simulink model "bev_motor_cooling"  (R2025a)
settings: Solver=VariableStepAuto  StartTime=0.0  StopTime=720  RelTol=1e-3  AbsTol=1e-3
PreLoadFcn:
  | bev_motor_cooling_param;
undefined symbols (not defined in the file): bev
libraries: fl_lib x24, SimscapeFluids_lib x4, nesl_utility x4, driver_maneuver_library x1, ee_lib x1, sdl_lib x1
CloseFcn:
  | try,close(h1_bev_motor_cooling),end
  | clear h1_bev_motor_cooling
  | try,close(h2_bev_motor_cooling),end
  | clear h2_bev_motor_cooling
  | try,close(h3_bev_motor_cooling),end
  | clear h3_bev_motor_cooling
  | try,close(h4_bev_motor_cooling),end
  | clear h4_bev_motor_cooling
  | 
  | 
  | clear simlog_bev_motor_cooling
  | clear logsout_bev_motor_cooling
Description:
  | Battery Electric Vehicle With Motor Cooling
  | 
  | 
  | Copyright 2021-2025 The MathWorks, Inc.
settings Model: Creator=kheintz  LastModifiedBy=smiller
settings SolverCC: AutoScaleAbsTol=off  AlgebraicLoopSolver=TrustRegion
settings DataIOCC: MaxDataPoints=10000  SignalLoggingName=logsout_bev_motor_cooling
settings OptimizationCC: ReuseModelBlockBuffer=off
settings DebuggingCC: UnconnectedInputMsg=warning  UnconnectedOutputMsg=warning  UnconnectedLineMsg=warning  SymbolicDimsDataTypeCodeGenerationDiagnostic=none
settings ModelReferenceCC: EnableRefExpFcnMdlSchedulingChecks=on
settings SFSimCC: CustomCodeUndefinedFunction=UseInterfaceOnly
settings RTWCC: GPUComputeCapability=3.5  DLArmComputeVersion=19.05
settings SimscapeCC: SimscapeLogType=all  SimscapeLogSimulationStatistics=on  SimscapeLogName=simlog_bev_motor_cooling  SimscapeLogDataHistory=10000.0

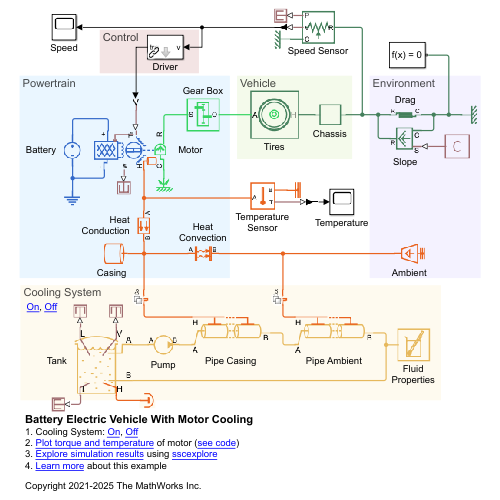
[thumbnail: Simulink's stored preview of the top-level diagram]
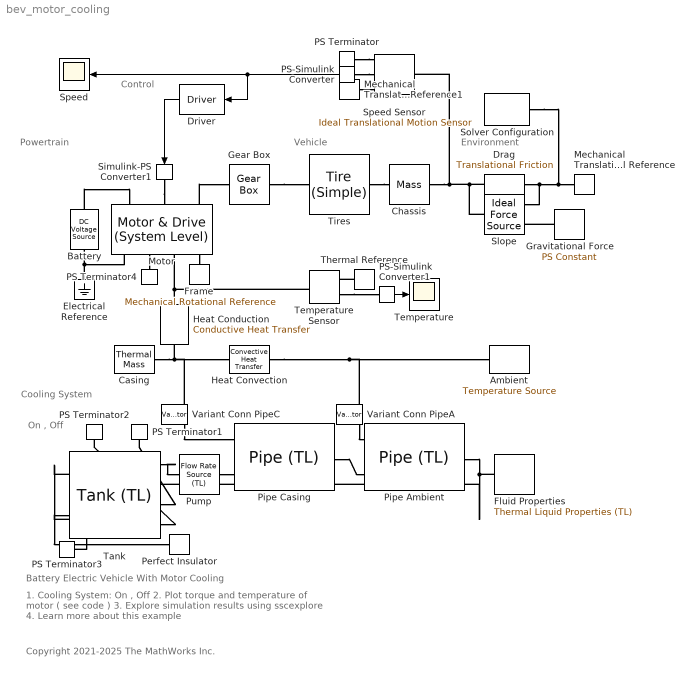
== system bev_motor_cooling ==
  note: Copyright 2021-2025 The MathWorks Inc.
  note: Control
  note: Environment
  note: Powertrain
  note: Vehicle
  note: Cooling System
  note: Battery Electric Vehicle With Motor Cooling
  note: 1. Cooling System: On , Off
      | 2. Plot torque and temperature of motor ( see code )
      | 3. Explore simulation results using sscexplore
      | 4. Learn more about this example
  note: On , Off
  Ambient : fl_lib/Thermal/Thermal Sources/Temperature Source  temperature=bev.Tambient degC
  Battery : fl_lib/Electrical/Electrical Sources/DC Voltage Source  v0=bev.battery.volt V
  Casing : fl_lib/Thermal/Thermal Elements/Thermal Mass  mass_type=foundation.enum.constant_variable.constant  mass=bev.casing.mass kg  sp_heat=bev.casing.sp_heat J/kg/K  mass_min=1e-6 kg  num_ports=foundation.enum.numPorts2.one  m_specify=off  m_priority=High  m=1 kg  m_nominal_specify=off  m_nominal_value=1  m_nominal_unit=kg  T_specify=on  T_priority=High  T=bev.casing.initT degC  T_nominal_specify=off  T_nominal_value=1  T_nominal_unit=K  Q_specify=off  Q_priority=None  Q=0 W  Q_nominal_specify=off  Q_nominal_value=1  Q_nominal_unit=W
  Chassis : fl_lib/Mechanical/Translational Elements/Mass  mass=bev.car.mass kg  num_ports=foundation.enum.numPorts2.two  v_specify=off  v_priority=Low  v=100 km/hr  v_nominal_specify=off  v_nominal_value=10  v_nominal_unit=m/s  f_specify=off  f_priority=None  f=0 N  f_nominal_specify=off  f_nominal_value=1  f_nominal_unit=N
      settings: InternalSimscapePortConfiguration="{\"Bottom\":[],\"Left\":[{\"id\":\"M\",\"label\":\"\",\"type\":\"foundation.mechanical.translational.translational\"}],\"Right\":[{\"id\":\"N\",\"label\":\"\",\"type\":\"foundation.mechanical.translational.translational\"}],\"Top\":[]}"
  Drag : fl_lib/Mechanical/Translational Elements/Translational Friction  brkwy_frc=bev.car.drag.brk N  brkwy_vel=bev.car.drag.vth m/s  Col_frc=bev.car.drag.fcl N  visc_coef=bev.car.drag.cvs N/(m/s)  v_specify=off  v_priority=None  v=0 m/s  v_nominal_specify=off  v_nominal_value=1  v_nominal_unit=m/s  f_specify=off  f_priority=None  f=0 N  f_nominal_specify=off  f_nominal_value=1  f_nominal_unit=N
      settings: InternalSimscapePortConfiguration="{\"Bottom\":[],\"Left\":[{\"id\":\"R\",\"label\":\"R\",\"type\":\"foundation.mechanical.translational.translational\"}],\"Right\":[{\"id\":\"C\",\"label\":\"C\",\"type\":\"foundation.mechanical.translational.translational\"}],\"Top\":[]}"
  Driver : driver_maneuver_library/Driver  max_torque=800  spd_cruise_1=100  spd_other_car=80  initial_lead_dist=100  follow_dist=40  pass_start_time=180  spd_passing=160  lead_dist=20  spd_cruise_2=100
  Electrical Reference : fl_lib/Electrical/Electrical Elements/Electrical Reference
  Fluid Properties : SimscapeFluids_lib/Thermal Liquid/Utilities/Thermal Liquid Properties (TL)  fluid_list=fluids.thermal_liquid.utilities.enum.thermal_liquid_fluid_list.ethylene_glycol  concentration_param_EG=fluids.thermal_liquid.utilities.enum.thermal_liquid_concentration.volume_fraction  concentration_param_PG=fluids.thermal_liquid.utilities.enum.thermal_liquid_concentration.volume_fraction  c_mass_SW=3.5e-3  c_mass_EG=0.1  c_mass_PG=0.1  c_mass_GL=0.1  c_vol_EG=0.5  c_vol_PG=0.1  beta_const_EG=2.1791 GPa  beta_const_PG=2.1791 GPa  beta_const_GL=2.1791 GPa  p_min_EG=0.01 MPa  p_min_PG=0.01 MPa  p_min_GL=0.01 MPa  p_max_EG=50 MPa  p_max_PG=50 MPa  p_max_GL=50 MPa  p_atm=0.101325 MPa  properties_range_check=simscape.enum.assert.action.error
  Frame : fl_lib/Mechanical/Rotational Elements/Mechanical Rotational Reference
  Gear Box : fl_lib/Mechanical/Mechanisms/Gear Box  Tag=varswap  ratio=bev.car.gear.rat  t_in_specify=off  t_in_priority=None  t_in=0 N*m  t_in_nominal_specify=off  t_in_nominal_value=1  t_in_nominal_unit=N*m  t_out_specify=off  t_out_priority=None  t_out=0 N*m  t_out_nominal_specify=off  t_out_nominal_value=1  t_out_nominal_unit=N*m
  Gravitational Force : fl_lib/Physical Signals/Sources/PS Constant  constant=bev.road.gforce N
  Heat Conduction : fl_lib/Thermal/Thermal Elements/Conductive Heat Transfer  thermal_type=foundation.enum.ConstantVariableTabulated.Constant  wall_geometry=foundation.enum.ConductionWallGeometry.Planar  area=bev.motor.qcond.area m^2  thickness=bev.motor.qcond.thick m  d_in=0.05 m  d_out=0.1 m  L=1 m  th_cond_min=10 W/(K*m)  th_cond=bev.motor.qcond.th_cond W/(m*K)  th_cond_TLU=[413, 401, 392, 383, 371, 357, 342] W/(K*m)  temp_TLU=[200, 273, 400, 600, 800, 1000, 1200] K  T_specify=off  T_priority=None  T=0 K  T_nominal_specify=off  T_nominal_value=1  T_nominal_unit=K  Q_specify=off  Q_priority=None  Q=1 W  Q_nominal_specify=off  Q_nominal_value=1  Q_nominal_unit=W
  Heat Convection : fl_lib/Thermal/Thermal Elements/Convective Heat Transfer  thermal_type=foundation.enum.constant_variable.constant  area=bev.casing.qconv.area m^2  heat_tr_coeff=bev.casing.qconv.th_conv W/(m^2 * K)  min_heat_tr_coeff=1e-3 W/(K*m^2)  T_specify=off  T_priority=None  T=0 K  T_nominal_specify=off  T_nominal_value=1  T_nominal_unit=K  Q_specify=off  Q_priority=None  Q=0 W  Q_nominal_specify=off  Q_nominal_value=1  Q_nominal_unit=W
  Mechanical Translational Reference : fl_lib/Mechanical/Translational Elements/Mechanical Translational Reference
  Mechanical Translational Reference1 : fl_lib/Mechanical/Translational Elements/Mechanical Translational Reference
  Motor : ee_lib/Electromechanical/Motor & Drive (System Level)  torque_speed_param=ee.enum.electromech.envelope.torque_power  overtorque_param=ee.enum.electromech.overtorque.no  T_t=[.09, .08, .07, 0] N*m  T_t_intermittent=[.36, .32, .28, 0] N*m  T_t_2D=[.09, .09, .09; .08, .08, .08; .07, .07, .07; 0, 0, 0] N*m  T_t_intermittent_2D=[.36, .36, .36; .32, .32, .32; .28, .28, .28; 0, 0, 0] N*m  w_t=[0, 3750, 7500, 8000] rpm  vdc_t=[6, 12, 24] V  torque_max=bev.motor.maxtrq N*m  power_max=bev.motor.maxpwr W  torque_max_intermittent=0.4 N*m  power_max_intermittent=120 W  time_overtorque=30 s  time_recover=60 s  Tc=bev.motor.tc s  EnableSwitch=simscape.enum.onoff.off  losses_param=1  eff=bev.motor.eff  w_eff=bev.motor.w_eff rpm  T_eff=bev.motor.T_eff N*m  Piron=bev.motor.Piron W  Pbase=bev.motor.Pbase W  w_eff_vec=[-8000, -4000, 0, 4000, 8000] rpm  T_eff_vec=[0, .03, .06, .09] N*m  v_eff_vec=[100, 250, 400] V  losses_mat=[1.49, 1.67, 2.21, 3.1; .42, .69, 1.14, 2.03; .06, .24, .78, 1.68; .42, .69, 1.14, 2.03; 1.49, 1.67, 2.21, 3.1] W  efficiency_mat=[95, 95, 95, 95; 95, 95, 95, 95; 95, 95, 95, 95; 95, 95, 95, 95; 95, 95, 95, 95]  losses_mat_3D=ones(5, 4, 3) W  efficiency_mat_3D=95 * ones(5, 4, 3)  Res=bev.motor.Res Ohm  J=bev.motor.J kg*m^2  lam=bev.motor.lam N*m/(rad/s)  speed0=bev.motor.speed0 rpm  faulted_specify=off  faulted_priority=None  faulted=0  faulted_nominal_specify=off  faulted_nominal_value=1  faulted_nominal_unit=1  isSwitchedOff_specify=off  isSwitchedOff_priority=None  isSwitchedOff=0  isSwitchedOff_nominal_specify=off  isSwitchedOff_nominal_value=1  isSwitchedOff_nominal_unit=1  torqueLimitContinuous_specify=off  torqueLimitContinuous_priority=None  torqueLimitContinuous=0 N*m  torqueLimitContinuous_nominal_specify=off  torqueLimitContinuous_nominal_value=1  torqueLimitContinuous_nominal_unit=N*m  alpha=bev.motor.alpha 1/K  Tmeas=bev.motor.Tmeas degC  Tmeas2=125 degC  losses_mat_T2=[1.49, 1.74, 2.49, 3.74; .42, .67, 1.42, 2.67; .06, .31, 1.06, 2.31; .42, .67, 1.42, 2.67; 1.49, 1.74, 2.49, 3.74] W  efficiency_mat_T2=[95, 95, 95, 95; 95, 95, 95, 95; 95, 95, 95, 95; 95, 95, 95, 95; 95, 95, 95, 95]  losses_mat_3D_T2=ones(5, 4, 3) W  efficiency_mat_3D_T2=95 * ones(5, 4, 3)  thermal_mass=bev.motor.thermal_mass J/K  initial_temperature=bev.motor.initT degC
      settings: InternalSimscapePortConfiguration="{\"Bottom\":[],\"Left\":[{\"id\":\"Vp\",\"label\":\"+\",\"type\":\"foundation.electrical.electrical\"},{\"id\":\"Tr\",\"label\":\"Tr\",\"type\":\"input\"},{\"id\":\"R\",\"label\":\"R\",\"type\":\"foundation.mechanical.rotational.rotational\"}],\"Right\":[{\"id\":\"Vm\",\"label\":\"-\",\"type\":\"foundation.electrical.electrical\"},{\"id\":\"Omega\",\"label\":\"w\",\"type\":\"output\"},{\"id\":\"H\",\"label\":\"H\",\"type\":\"foundation.thermal.thermal\"},{\"id\":\"C\",\"label\":\"C\",\"type\":\"foundation.mechanical.rotational.rotational\"}],\"Top\":[]}"
  PS Terminator{,1..4} (5 alike) : fl_lib/Physical Signals/Sinks/PS Terminator
  PS-Simulink Converter : nesl_utility/PS-Simulink Converter  PhysicalDomain=network_engine_domain  SubClassName=ps_output  LeftPortType=input  RightPortType=output  PseudoPeriodic=off  Frequencies=[]  VectorFormat=1-D array  Unit=km/hr  AffineConversion=off
  PS-Simulink Converter1 : nesl_utility/PS-Simulink Converter  PhysicalDomain=network_engine_domain  SubClassName=ps_output  LeftPortType=input  RightPortType=output  PseudoPeriodic=off  Frequencies=[]  VectorFormat=1-D array  Unit=degC  AffineConversion=on
  Perfect Insulator : fl_lib/Thermal/Thermal Elements/Perfect Insulator  T_specify=off  T_priority=None  T=0 K  T_nominal_specify=off  T_nominal_value=1  T_nominal_unit=K
  Pipe Ambient : SimscapeFluids_lib/Thermal Liquid/Pipes & Fittings/Pipe (TL)  dynamic_compressibility=1  inertia=0  num_segments=10  pipe_length=5 m  cross_section_geometry=fluids.thermal_liquid.pipes_fittings.enum.CrossSectionGeometry.Custom  pipe_diameter=0.1 m  pipe_inner_diameter=0.05 m  pipe_outer_diameter=0.1 m  pipe_width=0.1 m  pipe_height=0.1 m  pipe_major_axis=0.1 m  pipe_minor_axis=0.05 m  pipe_side=0.1 m  pipe_angle=30 deg  area=bev.cooling.area m^2  Dh=bev.cooling.hd m  elevation_spec=foundation.enum.constant_variable.constant  elevation_gain=0 m  gravity_spec=foundation.enum.constant_variable.constant  g=9.81 m/s^2  pressure_loss_spec=1  local_pressure_loss_spec=fluids.thermal_liquid.pipes_fittings.enum.LocalLossSpec.AggregateLength  length_add=1 m  loss_coefficient=0.1  roughness_spec=fluids.thermal_liquid.pipes_fittings.enum.RoughnessSpec.Custom  roughness=1.5e-5 m  Re_friction_TLU=[ 400 1000 1.5e+3 3e+3 4e+3 6e+3 1e+4 2e+4 4e+4 6e+4 1e+5 1e+8 ]  friction_factor_TLU=[ 0.264 0.112 0.07099999999999999 0.0417 0.0387 0.0268 0.025 0.0232 0.0226 0.022 0.0214 0.0214 ]  Re_lam=2e+3  Re_tur=4e+3  shape_factor=64  mdot_nominal=[ 0.1 1 ] kg/s  p_diff_nominal=[ 0.001 0.01 ] MPa  mdot_threshold=1e-6 kg/s  wall_spec=1  vol_expansion_spec=fluids.thermal_liquid.pipes_fittings.enum.VolumeExpansionSpec.Diameter  area_pressure_gain=1e-6 m^2/MPa  static_pressure_TLU=[.1, 1] MPa  area_pressure_gain_TLU=[1e-05, 1.1e-05] m^2  material_behavior_spec=fluids.thermal_liquid.pipes_fittings.enum.PipeMaterialBehavior.Linear  diameter_pressure_gain=1.2e-6 m/MPa  wall_thickness=0.05 m  elastic_modulus=69 GPa  stress_TLU=[276, 310] MPa  strain_TLU=[.004, .02]  stress_assert_action=simscape.enum.assert.action.none  stress_max=400 MPa  poisson_ratio=0.33  wall_time_constant=0.01 s  thermal_expansion=false  alpha_L_wall=24 um/(deltaK*m)  thermal_expansion_Tref=293.15 K  heat_transfer_spec=1  mdot_nominal_heat=[ 0.1 1 ] kg/s  T_in_nominal=[ 293.15 293.15 ] K  T_out_nominal=[ 300 300 ] K  p_in_nominal_heat=[ 0.101325 0.101325 ] MPa  T_wall_nominal=[ 303.15 303.15 ] K  a_coeff=0.023  b_Re_power=0.8  c_Pr_power=0.4  Nu_lam=3.66  Re_Colburn_TLU=[ 100 150 1000 ]  Colburn_factor_TLU=[ 0.019 0.013 0.002 ]  Re_Nu_TLU=[ 100 150 1000 ]  Pr_Nu_TLU=[ 1 10 ]  Nu_TLU=[ 3.72 4.21; 3.75 4.44; 4.21 7.15 ]  p0_vec=0.101325 MPa  T0_vec=bev.Tambient degC  mdot0=0.1 kg/s  p_nominal=0.101325 MPa  T_nominal=293.15 K
  Pipe Casing : SimscapeFluids_lib/Thermal Liquid/Pipes & Fittings/Pipe (TL)  dynamic_compressibility=1  inertia=0  num_segments=10  pipe_length=5 m  cross_section_geometry=fluids.thermal_liquid.pipes_fittings.enum.CrossSectionGeometry.Custom  pipe_diameter=0.1 m  pipe_inner_diameter=0.05 m  pipe_outer_diameter=0.1 m  pipe_width=0.1 m  pipe_height=0.1 m  pipe_major_axis=0.1 m  pipe_minor_axis=0.05 m  pipe_side=0.1 m  pipe_angle=30 deg  area=bev.cooling.area m^2  Dh=bev.cooling.hd m  elevation_spec=foundation.enum.constant_variable.constant  elevation_gain=0 m  gravity_spec=foundation.enum.constant_variable.constant  g=9.81 m/s^2  pressure_loss_spec=1  local_pressure_loss_spec=fluids.thermal_liquid.pipes_fittings.enum.LocalLossSpec.AggregateLength  length_add=1 m  loss_coefficient=0.1  roughness_spec=fluids.thermal_liquid.pipes_fittings.enum.RoughnessSpec.Custom  roughness=1.5e-5 m  Re_friction_TLU=[ 400 1000 1.5e+3 3e+3 4e+3 6e+3 1e+4 2e+4 4e+4 6e+4 1e+5 1e+8 ]  friction_factor_TLU=[ 0.264 0.112 0.07099999999999999 0.0417 0.0387 0.0268 0.025 0.0232 0.0226 0.022 0.0214 0.0214 ]  Re_lam=2e+3  Re_tur=4e+3  shape_factor=64  mdot_nominal=[ 0.1 1 ] kg/s  p_diff_nominal=[ 0.001 0.01 ] MPa  mdot_threshold=1e-6 kg/s  wall_spec=1  vol_expansion_spec=fluids.thermal_liquid.pipes_fittings.enum.VolumeExpansionSpec.Diameter  area_pressure_gain=1e-6 m^2/MPa  static_pressure_TLU=[.1, 1] MPa  area_pressure_gain_TLU=[1e-05, 1.1e-05] m^2  material_behavior_spec=fluids.thermal_liquid.pipes_fittings.enum.PipeMaterialBehavior.Linear  diameter_pressure_gain=1.2e-6 m/MPa  wall_thickness=0.05 m  elastic_modulus=69 GPa  stress_TLU=[276, 310] MPa  strain_TLU=[.004, .02]  stress_assert_action=simscape.enum.assert.action.none  stress_max=400 MPa  poisson_ratio=0.33  wall_time_constant=0.01 s  thermal_expansion=false  alpha_L_wall=24 um/(deltaK*m)  thermal_expansion_Tref=293.15 K  heat_transfer_spec=1  mdot_nominal_heat=[ 0.1 1 ] kg/s  T_in_nominal=[ 293.15 293.15 ] K  T_out_nominal=[ 300 300 ] K  p_in_nominal_heat=[ 0.101325 0.101325 ] MPa  T_wall_nominal=[ 303.15 303.15 ] K  a_coeff=0.023  b_Re_power=0.8  c_Pr_power=0.4  Nu_lam=3.66  Re_Colburn_TLU=[ 100 150 1000 ]  Colburn_factor_TLU=[ 0.019 0.013 0.002 ]  Re_Nu_TLU=[ 100 150 1000 ]  Pr_Nu_TLU=[ 1 10 ]  Nu_TLU=[ 3.72 4.21; 3.75 4.44; 4.21 7.15 ]  p0_vec=0.101325 MPa  T0_vec=bev.casing.initT degC  mdot0=0.1 kg/s  p_nominal=0.101325 MPa  T_nominal=293.15 K
  Pump : fl_lib/Thermal Liquid/Sources/Flow Rate Source (TL)  source_type=foundation.enum.constant_controlled.constant  flow_type=foundation.enum.mass_volumetric_flow.mass  mass_flow=2 kg/s  volumetric_flow=0 m^3/s  power_spec=foundation.enum.power_spec.isentropic  area=0.01 m^2
      settings: InternalSimscapePortConfiguration="{\"Bottom\":[],\"Left\":[{\"id\":\"A\",\"label\":\"A\",\"type\":\"foundation.thermal_liquid.thermal_liquid\"}],\"Right\":[{\"id\":\"B\",\"label\":\"B\",\"type\":\"foundation.thermal_liquid.thermal_liquid\"}],\"Top\":[]}"
  Simulink-PS Converter1 : nesl_utility/Simulink-PS Converter  PhysicalDomain=network_engine_domain  SubClassName=ps_input  LeftPortType=input  RightPortType=output  PseudoPeriodic=off  Frequencies=[]  NoiseDistribution=none  NoiseParameters=[]  Unit=N*m  AffineConversion=off  FilteringAndDerivatives=provide  SimscapeFilterOrder=1  InputFilterTimeConstant=0.001  UdotUserProvided=0
  Slope : fl_lib/Mechanical/Mechanical Sources/Ideal Force Source
  Solver Configuration : nesl_utility/Solver Configuration  PhysicalDomain=network_engine_domain  SubClassName=solver  LeftPortType=input  RightPortType=generic  Tones=[]  Harmonics=[]  SimulateNoise=off  Profile=off  UseLocalSampling=off  EnableSwitchedLinearOptims=on  FrequencyDomain=off  UseCCode=off  RelTol=0.001  AbsTol=1e-06  MinStep=1e-09  ToWorkspace=off  RevertToSquareIcSolve=off  NumHomotopyIterations=100  PhasorMode=off  PhasorModeNumHarmonics=1  ConsistencySolver=NEWTON_FTOL  IndexReductionMethod=DerivativeReplacement  DoDC=off  ResidualTolerance=1e-09  ConsistencyTolSource=GLOBAL  ConsistencyAbsTol=0.001  ConsistencyRelTol=0.001  ConsistencyTolFactor=0.001  UseLocalSolver=off  LocalSolverChoice=NE_BACKWARD_EULER_ADVANCER  ResolveIndetEquations=on  FunctionEvalNumThread=1  LocalSolverSampleTime=0.001  DoFixedCost=off  MaxNonlinIter=3  MaxModeIter=2  ComputeImpulses=off  ImpulseIterations=2  LinearAlgebra=auto  LinearAlgebraNumThread=0  EquationFormulation=NE_TIME_EF  DelaysMemoryBudget=1024  AutomaticFiltering=on  FilteringTimeConstant=0.001  PartitionStorageMethod=AS_NEEDED  PartitionMemoryBudget=1024  PartitionMethod=ROBUST  MultibodyUseLocalSolver=off  MultibodyLocalSolverChoice=ODE1  MultibodyLocalSolverSampleTime=0.001
  Speed : Scope
      settings: ActiveDisplayYMinimum=-17.93765  ActiveDisplayYMaximum=161.38831
  Speed Sensor : fl_lib/Mechanical/Mechanical Sensors/Ideal Translational Motion Sensor  reference=foundation.enum.MeasurementReference.difference  acceleration_port=false  velocity_port=true  position_port=true  offset=0 m
  Tank : SimscapeFluids_lib/Thermal Liquid/Tanks & Accumulators/Tank (TL)  num_inlet=2  pressure_spec=1  tank_pressure=0.101325 MPa  volume_spec=1  tank_area=bev.tank.csec m^2  level_TLU=[0, 3, 5] m  volume_TLU=[0, 4, 6] m^3  inlet_height_A=[.1] m  inlet_area_A=[.01] m^2  inlet_heights_AB=[0, 0] m  inlet_areas_AB=[.01, .01] m^2  inlet_heights_ABC=[.1, .05, 0] m  inlet_areas_ABC=[.01, .01, .01] m^2  inlet_heights_ABCD=linspace(0.1, 0, 4) m  inlet_areas_ABCD=0.01 * ones(1, 4) m^2  inlet_heights_ABCDE=linspace(0.1, 0, 5) m  inlet_areas_ABCDE=0.01 * ones(1, 5) m^2  inlet_heights_ABCDEF=linspace(0.1, 0, 6) m  inlet_areas_ABCDEF=0.01 * ones(1, 6) m^2  level_check=simscape.enum.assert.action.error  capacity_check=1  max_capacity=bev.tank.vol m^3  g=9.81 m/s^2  level_specify=on  level_priority=None  level=1 m  level_nominal_specify=off  level_nominal_value=1  level_nominal_unit=m  volume_specify=on  volume_priority=High  volume=bev.tank.volInit m^3  volume_nominal_specify=off  volume_nominal_value=1  volume_nominal_unit=m^3  mass_specify=off  mass_priority=None  mass=5e+3 kg  mass_nominal_specify=off  mass_nominal_value=1  mass_nominal_unit=kg  T_I_specify=on  T_I_priority=High  T_I=bev.Tambient degC  T_I_nominal_specify=off  T_I_nominal_value=1  T_I_nominal_unit=K
      settings: InternalSimscapePortConfiguration="{\"Bottom\":[{\"id\":\"H\",\"label\":\"H\",\"type\":\"foundation.thermal.thermal\"},{\"id\":\"T_out\",\"label\":\"T\",\"type\":\"output\"}],\"Left\":[{\"id\":\"A\",\"label\":\"A\",\"type\":\"foundation.thermal_liquid.thermal_liquid\"},{\"id\":\"B\",\"label\":\"B\",\"type\":\"foundation.thermal_liquid.thermal_liquid\"}],\"Right\":[],\"Top\":[{\"id\":\"V_out\",\"label\":\"V\",\"type\":\"output\"},{\"id\":\"L_out\",\"label\":\"L\",\"type\":\"output\"}]}"
  Temperature : Scope
      settings: ActiveDisplayYMinimum=32.57224  ActiveDisplayYMaximum=190.78819
  Temperature Sensor : fl_lib/Thermal/Thermal Sensors/Temperature Sensor  temperature_measure=foundation.enum.MeasurementReference.difference
  Thermal Reference : fl_lib/Thermal/Thermal Elements/Thermal Reference
  Tires : sdl_lib/Tires & Vehicles/Tire (Simple)  r_tire=bev.car.tire.rad cm  model_compliance=0  stiffness=1e6 N/m  damping=1000 N/(m/s)  model_inertia=0  tire_inertia=1 kg*m^2  initial_velocity=0 rad/s
      settings: InternalSimscapePortConfiguration="{\"Bottom\":[],\"Left\":[{\"id\":\"A\",\"label\":\"A\",\"type\":\"foundation.mechanical.rotational.rotational\"}],\"Right\":[{\"id\":\"H\",\"label\":\"H\",\"type\":\"foundation.mechanical.translational.translational\"}],\"Top\":[]}"
  Variant Conn PipeA : VariantPMConnector  ConnectorBlkType=Nonprimary  ConnectorTag=Cool
  Variant Conn PipeC : VariantPMConnector  VariantControls=__PRM__SERIALIZED__DATA__:Cooling_On==1  ConnectorBlkType=Primary  ConnectorTag=Cool
  wires:
  PS-Simulink Converter1/1 -> Temperature/1
  Driver/1 -> Simulink-PS Converter1/1
  PS-Simulink Converter/1 -> Driver/1, Speed/1
  connections:
  Variant Conn PipeA/LConn1 -- Pipe Ambient/LConn2
  Temperature Sensor/LConn1 -- Motor/RConn3 -- Heat Conduction/LConn1
  Drag/LConn1 -- Slope/LConn1 -- Chassis/RConn1 -- Speed Sensor/LConn1
  Drag/RConn1 -- Slope/RConn2 -- Mechanical Translational Reference/LConn1 -- Solver Configuration/RConn1
  Electrical Reference/LConn1 -- Motor/RConn1 -- Battery/RConn1
  Fluid Properties/RConn1 -- Tank/LConn2 -- Pipe Ambient/RConn1
  Simulink-PS Converter1/RConn1 -- Motor/LConn2
  Pipe Casing/RConn1 -- Pipe Ambient/LConn1
  Pump/RConn1 -- Pipe Casing/LConn1
  Temperature Sensor/RConn2 -- PS-Simulink Converter1/LConn1
  Motor/LConn3 -- Gear Box/LConn1
  Mechanical Translational Reference1/LConn1 -- Speed Sensor/RConn1
  PS-Simulink Converter/LConn1 -- Speed Sensor/RConn2
  Gravitational Force/RConn1 -- Slope/RConn1
  Tank/LConn1 -- Pump/LConn1
  Battery/LConn1 -- Motor/LConn1
  Thermal Reference/LConn1 -- Temperature Sensor/RConn1
  Gear Box/RConn1 -- Tires/LConn1
  Motor/RConn4 -- Frame/LConn1
  Tires/RConn1 -- Chassis/LConn1
  PS Terminator/LConn1 -- Speed Sensor/RConn3
  Casing/LConn1 -- Heat Convection/LConn1 -- Variant Conn PipeC/RConn1 -- Heat Conduction/RConn1
  Variant Conn PipeC/LConn1 -- Pipe Casing/LConn2
  Heat Convection/RConn1 -- Variant Conn PipeA/RConn1 -- Ambient/LConn1
  Motor/RConn2 -- PS Terminator4/LConn1
  Tank/LConn3 -- PS Terminator1/LConn1
  Tank/LConn4 -- PS Terminator2/LConn1
  Tank/RConn2 -- PS Terminator3/LConn1
  Tank/RConn1 -- Perfect Insulator/LConn1
